simulink model "tdpReplay"  (R2026b)
settings: Solver=FixedStepDiscrete  StopTime=2  FixedStep=P.dt
model workspace (MAT data in the model file):
  P.L = 9
  P.W = 6
  P.goalD = 0.6
  P.goalW = 2.6
  P.goalAreaL = 1
  P.goalAreaW = 3
  P.penMark = 1.5
  P.centreD = 1.5
  P.border = 1
  P.penAreaL = 2
  P.penAreaW = 5
  P.ballR = 0.07
  P.ballDecel = 0.4
  P.ballRestit = 0.5
  P.ballRobotE = 0.3
  P.robotR = 0.15
  P.vFwd = 0.25
  P.vBack = 0.12
  P.vSide = 0.15
  P.wMax = 0.785398163397
  P.Kp = 0.8
  P.Kw = 2
  P.avoidR = 0.7
  P.avoidGain = 0.6
  P.ballAvoidR = 0.35
  P.approachDist = 0.45
  P.kickRange = 0.28
  P.stepInSpeed = 0.1
  P.kickAlign = 0.349065850399
  P.behindTol = 0.523598775598
  P.kickNoise = 0.10471975512
  P.kickCooldown = 1
  P.shotSpeed = 1.8
  P.dribbleSpeed = 0.6
  P.maxKickSpeed = 2.2
  P.roleHyst = 0.4
  P.shootDist = 3
  P.defDist = 1.8
  P.nPerTeam = 4
  P.dt = 0.05
  P.Tmatch = 600
  P.restartPause = 2
  P.outPause = 1
  P.drawEvery = 4
  P.realtime = 0
  P.dirSign = [1 -1]
  P.seed = 1
  P.mode : TdpMode (value not decoded)
  P.rulesProfile : TdpRules (value not decoded)
  P.maxObservationAge = 0.5
  P.walkValidity = 0.1
  P.kickPreparation = 0.2
  P.kickTimeout = 1
  P.recoverTime = 0.5
  P.alignEnter = 0.35
  P.alignExit = 0.45
  P.searchTurnRate = 0.3
  P.fieldOfView = 6.28318530718
  P.observationDelay = 0
  P.observationNoise = 0
  P.fixedStriker = 0
  P.tapSpeed = 0.3
  P.freezeDuringPause = 0
  P.contactIterations = 256
  P.restartOpponentDistance = 0.75
  P.contactTolerance = 1e-10
  scenario : object (value not decoded)
symbols that are objects in the model workspace (value not decoded): scenario
libraries: ControllerCore x1
settings Model: DataDictionary=TdpTypes.sldd  Creator=fayne  LastModifiedBy=fayne
settings DataIOCC: SaveOutput=off  SignalLogging=off
settings DebuggingCC: AlgebraicLoopMsg=error

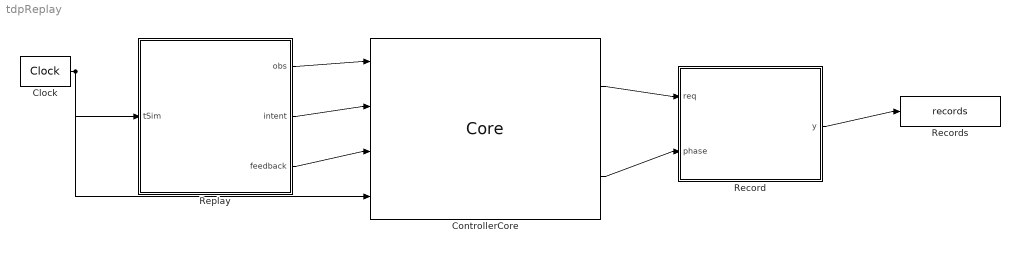
== system tdpReplay ==
  Clock : DigitalClock  SampleTime=P.dt
  ControllerCore : ControllerCore/Core  SystemSampleTime=-1  VariantActivationTime=update diagram  EmptyChoice=off  PassThrough=off  PassThroughVariantControl=(default)  EmptyChoiceVariantControl=(default)  AllowFlexibleInterface=on  Latency=0  AutoFrameSizeCalculation=off
  Record : MATLAB Function  TreatAsAtomicUnit=on
  Records : ToWorkspace  VariableName=records  SampleTime=-1
  Replay : MATLAB Function  TreatAsAtomicUnit=on
  wires:
  Replay/1(obs) -> ControllerCore/1
  Replay/2(intent) -> ControllerCore/2
  Replay/3(feedback) -> ControllerCore/3
  Clock/1 -> Replay/1(tSim), ControllerCore/4
  ControllerCore/1 -> Record/1(req)
  ControllerCore/2 -> Record/2(phase)
  Record/1(y) -> Records/1

== matlab function tdpReplay/Record ==
  data: req input Bus: RequestBus; y output; phase input Enum: TdpPhase
function y=f(req,phase)
y=[double(req.kind) double(req.requestId) double(phase) req.velocity req.target req.speed req.stamp req.validUntil];
end

== matlab function tdpReplay/Replay ==
  data: tSim input; obs output Bus: ObservationBus; intent output Bus: IntentBus; feedback output Bus: FeedbackBus; scenario parameter; P parameter
function [obs,intent,feedback]=f(tSim,scenario, P)
k=min(numel(scenario),max(1,round(tSim/P.dt)+1));
obs=scenario(k).obs;intent=scenario(k).intent;feedback=scenario(k).feedback;
end
